simulink model "IPMSMAxleDriveEV_fihPedals"  (R2024a)
settings: Solver=FixedStepDiscrete  StartTime=0.0  StopTime=5  FixedStep=Ts  RelTol=1e-3  EnableMultiTasking=on
PreLoadFcn:
  | IPMSMAxleDriveEVData;
undefined symbols (not defined in the file): AL, Cd, cr1, cr2, g, i_t, Ld, Lq, Mv, p, psim, rho_a, Rw, Tmax, Ts, VDC_VECT
libraries: fl_lib x40, nesl_utility x16, ee_lib x4, eeTransforms x2, simulink x2, batteryecm_lib x1, eePmsmCurrentController x1, eePmsmCurrentReferenceGen x1, eePmsmTorqueEstimator x1, eePwmGeneratorTwoLevel x1, SignalEditorBlockLib x1
CloseFcn:
  | try,close(h1_IPMSMAxleDriveEV),end
  | clear h1_IPMSMAxleDriveEV
  | 
  | clear simlog_IPMSMAxleDriveEV
  | clear logsout_IPMSMAxleDriveEV
  | 
  | 
  | clear Pmax Tmax p psim Ld Lq L0 Rs Jm
  | clear Cdc Vnom V1 AH0
  | clear Ts fsw Tsi Kp_id Ki_id Kp_iq Ki_iq
  | clear numd_id dend_id numd_iq dend_iq
  | clear ID_MAP IQ_MAP RPM_VECT TQ_VECT VDC_VECT
  | clear Mv g rho_a AL Cd cr1 cr2 i_t Rw
Description:
  | IPMSM Torque Control in an Axle-Drive EV
settings Model: Creator=The MathWorks, Inc.  LastModifiedBy=hirah
settings SolverCC: AlgebraicLoopSolver=TrustRegion  MaxZcPerStep=1
settings DataIOCC: MaxDataPoints=510000  ReturnWorkspaceOutputs=off  SignalLoggingName=logsout_IPMSMAxleDriveEV
settings OptimizationCC: ReuseModelBlockBuffer=off  LifeSpan=inf
settings DebuggingCC: UnderspecifiedInitializationDetection=Classic  MergeDetectMultiDrivingBlocksExec=none  UnconnectedInputMsg=warning  UnconnectedOutputMsg=warning  UnconnectedLineMsg=warning  SFUnexpectedBacktrackingDiag=warning  SFNoUnconditionalDefaultTransitionDiag=warning  SFExecutionAtInitializationDiag=none  ArithmeticOperatorsInVariantConditions=warning
settings ModelReferenceCC: EnableRefExpFcnMdlSchedulingChecks=on
settings SFSimCC: SimUseLocalCustomCode=off  CustomCodeUndefinedFunction=UseInterfaceOnly
settings RTWCC: RTWUseLocalCustomCode=off  GPUComputeCapability=3.5  DLArmComputeVersion=19.05
settings CodeAppCC: StateflowObjectComments=on
settings GRTTargetCC: TargetLangStandard=C89/C90 (ANSI)
settings ConfigComp: CovMetricSettings=dw  CovSaveCumulativeToWorkspaceVar=on  CovSaveSingleToWorkspaceVar=on  CovExternalEMLEnable=off
settings SimscapeCC: SimscapeNormalizeSystem=off  SimscapeLogType=all  SimscapeLogSimulationStatistics=on  SimscapeLogName=simlog_IPMSMAxleDriveEV  SimscapeLogDataHistory=510000

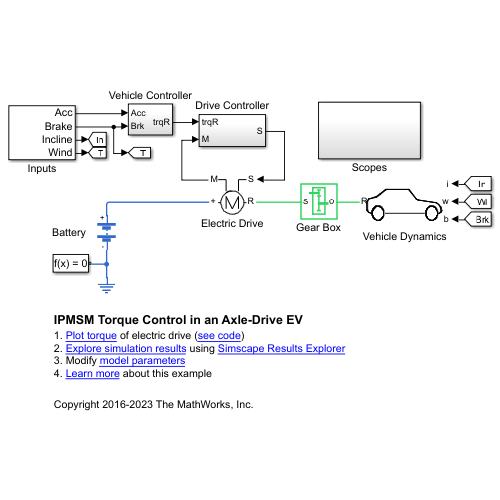
[thumbnail: Simulink's stored preview of the top-level diagram]
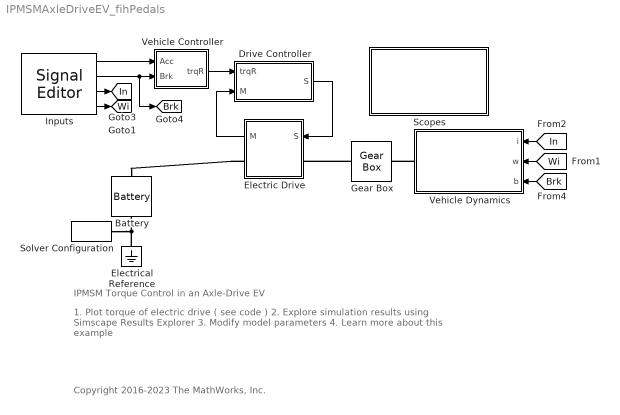
== system IPMSMAxleDriveEV_fihPedals ==
  note: IPMSM Torque Control in an Axle-Drive EV
  note: 1. Plot torque of electric drive ( see code )
      | 2. Explore simulation results using Simscape Results Explorer
      | 3. Modify model parameters
      | 4. Learn more about this example
  note: Copyright 2016-2023 The MathWorks, Inc.
  Battery : batteryecm_lib/Battery  Vnom=Vnom V  prm_dir=1  R1_dis=2 Ohm  R1_ch=2 Ohm  R1=0.001 Ohm  prm_AH=1  AH=300 hr*A  V1=V1 V  AH1=100 hr*A  prm_R2=1  R2=2000 Ohm  Tmeas=298.15 K  charge_measurement_port=simscape.enum.battery.enable.no  prm_dyn=1  Rp1=0.005 Ohm  tau1=30 s  Rp2=0.005 Ohm  tau2=30 s  Rp3=0.005 Ohm  tau3=30 s  Rp4=0.005 Ohm  tau4=30 s  Rp5=0.005 Ohm  tau5=30 s  prm_fade=1  N_fade=100  AH_fade=45 hr*A  R1_fade=2.02 Ohm  R1_ch_fade=2.02 Ohm  V1_fade=10.35 V  prm_age=1  prm_age_OCV=1  OCV_age=0.9  SOC_age=60  Tmeas_age=298.15 K  delta_time_age_vec=[0] d  temperature_age_vec=[273] K  OCV_scaling_age=2.2134e6  OCV_offset_age=1.632e6  temp_exp_age=0.515833569 V  t_exp_age=0.75  Vnom_T2=12 V  R1_T2=2.2 Ohm  R1_T2_dis=2.2 Ohm  R1_T2_ch=2.2 Ohm  V1_T2=11.4 V  R2_T2=2200 Ohm  Rp1_T2=0.005 Ohm  tau1_T2=30 s  Rp2_T2=0.005 Ohm  tau2_T2=30 s  Rp3_T2=0.005 Ohm  tau3_T2=30 s  Rp4_T2=0.005 Ohm  tau4_T2=30 s  Rp5_T2=0.005 Ohm  tau5_T2=30 s  Tmeas2=273.15 K  thermal_port=simscape.enum.thermaleffects.omit  thermal_mass=30000 J/K  i_specify=off  i_priority=None  i=0 A  i_nominal_specify=off  i_nominal_value=1  i_nominal_unit=A  v_specify=off  v_priority=None  v=0 V  v_nominal_specify=off  v_nominal_value=1  v_nominal_unit=V  charge_specify=on  charge_priority=High  charge=AH0 hr*A  charge_nominal_specify=off  charge_nominal_value=1  charge_nominal_unit=A*hr  num_cycles_specify=off  num_cycles_priority=High  num_cycles=0  num_cycles_nominal_specify=off  num_cycles_nominal_value=1  num_cycles_nominal_unit=1  temperature_specify=off  temperature_priority=High  temperature=298.15 K  temperature_nominal_specify=off  temperature_nominal_value=1  temperature_nominal_unit=K
  Drive Controller : Subsystem
  Electric Drive : Subsystem  Tag=PublishSubsystem
      mask Display:
      | % Circle
      | plot(sin(0:0.1:2.2*pi)*0.9,cos(0:0.1:2.2*pi)*0.9);
      | 
      | % In/out
      | plot([-1.1 -0.9],[0 0]);
      | plot([1.1 0.9],[0 0]);
      | 
      | % 'M'
      | plot([0.5 0.5],[-0.5 0.5]);
      | plot([-0.5 -0.5],[-0.5 0.5]);
      | plot([0.5 0],[0.5 -0.5]);
      | plot([-0.5 0],[0.5 -0.5]);
      | 
      | % Inputs and Outputs
      | plot([0.5 0.5],[0.9 1.8]);
      | plot([0.5 1.1],[1.8 1.8]);
      | 
      | plot([-0.5 -0.5],[0.9 1.8]);
      | plot([-0.5 -1.1],[1.8 1.8]);
      | 
      | 
      | % Plot points to set plot range
      | color('white');plot(1.9,2.8);plot(-1.9,0)
      | color('black');
  Electrical Reference : fl_lib/Electrical/Electrical Elements/Electrical Reference
  Gear Box : fl_lib/Mechanical/Mechanisms/Gear Box  ratio=i_t  t_in_specify=off  t_in_priority=None  t_in=0 N*m  t_in_nominal_specify=off  t_in_nominal_value=1  t_in_nominal_unit=N*m  t_out_specify=off  t_out_priority=None  t_out=0 N*m  t_out_nominal_specify=off  t_out_nominal_value=1  t_out_nominal_unit=N*m
  Inputs : SignalEditorBlockLib/Signal Editor  FileName=IPMSMAxleDriveEVInputs.mat  ActiveScenario=StartStop  ActiveSignal=Wind  IsBus=off  OutputBusObjectStr=Bus: BusObject  SampleTime=0  OutputAfterFinalValue=Extrapolation  Unit=inherit  PreserveSignalName=on  ApplySigPropsToAllScenarios=on  ApplySigPropsToAllSignals=off
  Scopes : Subsystem
  Solver Configuration : nesl_utility/Solver Configuration  PhysicalDomain=network_engine_domain  SubClassName=solver  LeftPortType=input  RightPortType=generic  Tones=[]  Harmonics=[]  SimulateNoise=off  Profile=off  UseLocalSampling=off  EnableSwitchedLinearOptims=on  FrequencyDomain=off  UseCCode=off  RelTol=0.001  AbsTol=1e-06  MinStep=1e-09  ToWorkspace=off  RevertToSquareIcSolve=off  NumHomotopyIterations=100  PhasorMode=off  PhasorModeNumHarmonics=1  ConsistencySolver=NEWTON_FTOL  IndexReductionMethod=DerivativeReplacement  DoDC=off  ResidualTolerance=1e-9  ConsistencyTolSource=GLOBAL  ConsistencyAbsTol=0.001  ConsistencyRelTol=0.001  ConsistencyTolFactor=0.001  UseLocalSolver=on  LocalSolverChoice=NE_BACKWARD_EULER_ADVANCER  ResolveIndetEquations=on  FunctionEvalNumThread=1  LocalSolverSampleTime=Ts  DoFixedCost=on  MaxNonlinIter=5  MaxModeIter=2  ComputeImpulses=off  ImpulseIterations=1  LinearAlgebra=auto  LinearAlgebraNumThread=0  EquationFormulation=NE_TIME_EF  DelaysMemoryBudget=1024  AutomaticFiltering=on  FilteringTimeConstant=0.001  PartitionStorageMethod=AS_NEEDED  PartitionMemoryBudget=1024  PartitionMethod=FAST  MultibodyUseLocalSolver=off  MultibodyLocalSolverChoice=ODE1  MultibodyLocalSolverSampleTime=0.001
  Vehicle Controller : Subsystem
  Vehicle Dynamics : Subsystem
      mask Display:
      | color('white')
      | plot(-120,-60); plot(120,50);
      | color('black')
      | plot(sin(0:0.1:6*pi)*15-70,cos(0:0.1:6*pi)*15-30);
      | plot(sin(0:0.1:6*pi)*15+70,cos(0:0.1:6*pi)*15-30);
      | plot([-88 -95 -99 -99 -95 -75 -65 -50 -46 10 30 34 80 85 90 93 95 93 90 88],[-30 -28 -23 -5 0 5 10 20 21 21 0 -2 -7 -9 -13 -17 -25 -28 -30 -30])
      | plot([-88 -95 -99 -99 -95 -75 -65 -50 -46 10 30 34 80 85 90 93 95 93 90 88],[-30 -28 -23 -5 0 5 10 20 21 21 0 -2 -7 -9 -13 -17 -25 -28 -30 -30]-1)
      | plot([-88 -95 -99 -99 -95 -75 -65 -50 -46 10 30 34 80 85 90 93 95 93 90 88]+1,[-30 -28 -23 -5 0 5 10 20 21 21 0 -2 -7 -9 -13 -17 -25 -28 -30 -30])
      | plot([-50 50],[-30 -30])
  tag scope: Brk=global, In=global, Wi=global
  wires:
  Vehicle Controller/1(trqR) -> Drive Controller/1(trqR)
  Electric Drive/1(M) -> Drive Controller/2(M)
  [Wi] -> Vehicle Dynamics/2(w)
  Drive Controller/1(S) -> Electric Drive/1(S)
  Inputs/3 -> [In]
  [Brk] -> Vehicle Dynamics/3(b)
  [In] -> Vehicle Dynamics/1(i)
  Inputs/1 -> Vehicle Controller/1(Acc)
  Inputs/2 -> [Brk], Vehicle Controller/2(Brk)
  Inputs/4 -> [Wi]
  connections:
  Battery/RConn1 -- Electrical Reference/LConn1 -- Solver Configuration/RConn1
  Electric Drive/RConn1 -- Battery/LConn1
  Gear Box/LConn1 -- Electric Drive/LConn1
  Vehicle Dynamics/RConn1 -- Gear Box/RConn1

== system IPMSMAxleDriveEV_fihPedals/Drive Controller ==
  trqR : Inport
  M : Inport  Port=2
  Bus Selector : BusSelector  OutputSignals=iabc,w,A,vdc
  EM Controller : Subsystem
  S : Outport  VectorParamsAs1DForOutWhenUnconnected=off
  wires:
  M/1 -> Bus Selector/1
  trqR/1 -> EM Controller/1(trqR)
  Bus Selector/1 -> EM Controller/2(iabc_sens)  "<iabc>"
  Bus Selector/2 -> EM Controller/3(w_sens)  "<w>"
  Bus Selector/3 -> EM Controller/4(th_sens)  "<A>"
  Bus Selector/4 -> EM Controller/5(Vdc_sens)  "<vdc>"
  EM Controller/1(S) -> S/1

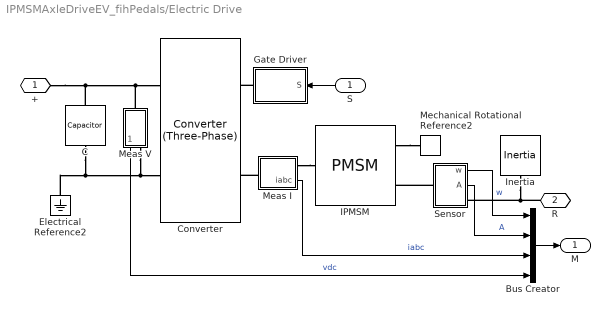
== system IPMSMAxleDriveEV_fihPedals/Electric Drive ==
  S : Inport
  Bus Creator : BusCreator  Inputs=4
  C : fl_lib/Electrical/Electrical Elements/Capacitor  c=Cdc F  r=1e-6 Ohm  g=0 1/Ohm  i_specify=off  i_priority=None  i=0 A  i_nominal_specify=off  i_nominal_value=1  i_nominal_unit=A  v_specify=off  v_priority=None  v=0 V  v_nominal_specify=off  v_nominal_value=1  v_nominal_unit=V  vc_specify=on  vc_priority=None  vc=Vnom V  vc_nominal_specify=off  vc_nominal_value=1  vc_nominal_unit=V
  Converter : ee_lib/Semiconductors & Converters/Converters/Converter (Three-Phase)  port_option=ee.enum.threePhasePort.composite  fidelity_option=ee.enum.converters.fidelity.detailed  device_type=3  K=0  Vf=0.8 V  Ron=0.001 Ohm  Rds=0.001 Ohm  Goff=1e-5 1/Ohm  Vgt=1 V  Vgt_off=-1 V  Ih=1 A  Vth=0.5 V  diode_param=2  diode_Vf=0.8 V  diode_Ron=0.001 Ohm  diode_Goff=1e-5 1/Ohm  diode_C=50 nF  diode_iRM=-235 A  diode_iF=300 A  diode_idot=-50 A/us  diode_trr_param=1  diode_trr_factor=3  diode_trr=15 us  diode_Qrr=1.5e+3 s*uA  snubber_type=0  Cs=1e-7 F  Rs=0.1 Ohm
  Electrical Reference2 : fl_lib/Electrical/Electrical Elements/Electrical Reference
  Gate Driver : Subsystem
  IPMSM : ee_lib/Electromechanical/Permanent Magnet/PMSM  port_option=ee.enum.threePhasePort.composite  winding_type=ee.enum.statorconnection.wye  machine_param=ee.enum.pmsm.parameterization.constant  nPolePairs=p  pmflux_param=1  pm_flux_linkage=psim Wb  torque_constant=0.18 N*m/A  back_emf_constant=0.18 V/(rad/s)  stator_param=1  Ld=Ld H  Lq=Lq H  idVec=[-200, 0, 200] A  iqVec=[-200, 0, 200] A  LdMatrix=0.0002 * ones(3, 3) H  LqMatrix=0.0002 * ones(3, 3) H  PmMatrix=0.1 * ones(3, 3) Wb  ktMatrix=0.18 * ones(3, 3) N*m/A  keMatrix=0.18 * ones(3, 3) V/(rad/s)  L0=L0 H  Ls=0.0002 H  Lm=0.00002 H  Ms=0.00002 H  Rs=Rs Ohm  zero_sequence=ee.enum.park.zerosequence.exclude  axes_param=1  loss_param=ee.enum.ironloss.none  losses_oc=[0, 0, 0] W  losses_sc=[0, 0, 0] W  f_losses=60 Hz  Isc_losses=95 A  J=0 kg*m^2  lam=0 N*m/(rad/s)  i_d_specify=off  i_d_priority=None  i_d=0 A  i_d_nominal_specify=off  i_d_nominal_value=1  i_d_nominal_unit=A  i_q_specify=off  i_q_priority=None  i_q=0 A  i_q_nominal_specify=off  i_q_nominal_value=1  i_q_nominal_unit=A  torque_specify=off  torque_priority=None  torque=0 N*m  torque_nominal_specify=off  torque_nominal_value=1  torque_nominal_unit=N*m  angular_velocity_specify=on  angular_velocity_priority=None  angular_velocity=0 rpm  angular_velocity_nominal_specify=off  angular_velocity_nominal_value=1  angular_velocity_nominal_unit=rpm  angular_position_specify=off  angular_position_priority=None  angular_position=0 deg  angular_position_nominal_specify=off  angular_position_nominal_value=1  angular_position_nominal_unit=deg  alpha=3.93e-3 1/K  alpha_flux=-0.001 1/K  Tmeas=298.15 K  stator_thermal_mass=100 J/K  rotor_thermal_mass=200 J/K  Rm_percent_rotor=90  Rd_percent_rotor=30  temperatureA_specify=off  temperatureA_priority=High  temperatureA=25 degC  temperatureA_nominal_specify=off  temperatureA_nominal_value=1  temperatureA_nominal_unit=degC  temperatureB_specify=off  temperatureB_priority=High  temperatureB=25 degC  temperatureB_nominal_specify=off  temperatureB_nominal_value=1  temperatureB_nominal_unit=degC  temperatureC_specify=off  temperatureC_priority=High  temperatureC=25 degC  temperatureC_nominal_specify=off  temperatureC_nominal_value=1  temperatureC_nominal_unit=degC  temperatureR_specify=off  temperatureR_priority=High  temperatureR=25 degC  temperatureR_nominal_specify=off  temperatureR_nominal_value=1  temperatureR_nominal_unit=degC
      settings: AttributesFormatString=35 kW  InternalSimscapePortConfiguration="{\"Bottom\":[],\"Left\":[{\"id\":\"N\",\"label\":\"~\",\"type\":\"foundation.electrical.three_phase\"}],\"Right\":[{\"id\":\"R\",\"label\":\"R\",\"type\":\"foundation.mechanical.rotational.rotational\"},{\"id\":\"C\",\"label\":\"C\",\"type\":\"foundation.mechanical.rotational.rotational\"}],\"Top\":[]}"
  Inertia : fl_lib/Mechanical/Rotational Elements/Inertia  inertia=Jm kg*m^2  num_ports=foundation.enum.numPorts2.one  w_specify=off  w_priority=High  w=0 rad/s  w_nominal_specify=off  w_nominal_value=1  w_nominal_unit=rad/s  t_specify=off  t_priority=None  t=0 N*m  t_nominal_specify=off  t_nominal_value=1  t_nominal_unit=N*m
  Meas I : Subsystem
      settings: PortSchema="{\"entries\":[{\"content\":{\"sides\":[{\"content\":{\"connectorIds\":[\"LConn1\"]},\"type\":\"ConnectorPlacement.EquallySpacedRectSide\",\"uuid\":\"3a4028b2-8937-42a6-80f4-68b1695ce77d\"},{\"content\":{\"connectorIds\":[\"RConn1\",\"Out1\"],\"side\":\"RIGHT\"},\"type\":\"ConnectorPlacement.EquallySpacedRectSide\",\"uuid\":\"b0265b90-0b10-444b-91c2-8367167e2f75\"},{\"content\":{\"connectorIds\":[],\"side\":\"TOP\"},\"type\":\"ConnectorPlacement.EquallySpacedRectSide\",\"uuid\":\"a56d3a18-e083-4f19-8a6c-1d5eb0dcfc62\"}]},\"type\":\"ConnectorPlacement.EquallySpacedConnector\",\"uuid\":\"f333dc84-7c1b-47f0-a9ed-bc0e1c61b934\"}],\"packageUris\":[\"http://schema.mathworks.com/mf0/Connector/R2020b\"],\"version\":\"1.0\"}"
      mask Display: %disp('iABC');
  Meas V : Subsystem
  Mechanical Rotational Reference2 : fl_lib/Mechanical/Rotational Elements/Mechanical Rotational Reference
  Sensor : Subsystem
  + : PMIOPort  Side=Right
  R : PMIOPort  Port=2  Side=Left
  M : Outport  VectorParamsAs1DForOutWhenUnconnected=off
  wires:
  S/1 -> Gate Driver/1(S)
  Bus Creator/1 -> M/1
  Meas I/1(iabc) -> Bus Creator/3  "iabc"
  Sensor/1(w) -> Bus Creator/1  "w"
  Sensor/2(A) -> Bus Creator/2  "A"
  Meas V/1(Vdc) -> Bus Creator/4  "vdc"
  connections:
  Gate Driver/RConn1 -- Converter/LConn1
  IPMSM/RConn2 -- Mechanical Rotational Reference2/LConn1
  Meas I/LConn1 -- Converter/LConn2
  Sensor/LConn1 -- IPMSM/RConn1
  Meas I/RConn1 -- IPMSM/LConn1
  R/RConn1 -- Sensor/RConn1 -- Inertia/LConn1
  +/RConn1 -- C/LConn1 -- Meas V/LConn1 -- Converter/RConn1
  Electrical Reference2/LConn1 -- C/RConn1 -- Meas V/RConn1 -- Converter/RConn2

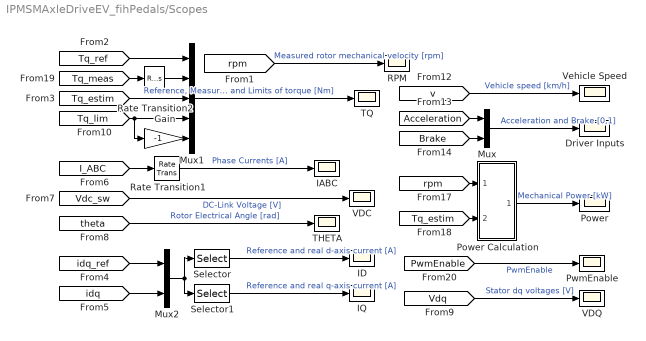
== system IPMSMAxleDriveEV_fihPedals/Scopes ==
  Driver Inputs : Scope
  Gain : Gain  Gain=-1
  IABC : Scope
  ID : Scope
  IQ : Scope
  Mux : Mux  Inputs=2
  Mux1 : Mux  Inputs=5
  Mux2 : Mux  Inputs=2
  Power : Scope
  Power Calculation : Subsystem
  PwmEnable : Scope
  RPM : Scope
  Rate Transition1 : RateTransition  OutPortSampleTime=1e-4
  Rate Transition2 : RateTransition
  Selector : Selector  InputPortWidth=4  IndexOptions=Index vector (dialog)  Indices=[1 3]  OutputSizes=1
  Selector1 : Selector  InputPortWidth=4  IndexOptions=Index vector (dialog)  Indices=[2 4]  OutputSizes=1
  THETA : Scope
  TQ : Scope
  VDC : Scope
  VDQ : Scope
  Vehicle Speed : Scope
  wires:
  Power Calculation/1(Power) -> Power/1  "Mechanical Power [kW]"
  Gain/1 -> Mux1/5
  [idq] -> Mux2/2
  [Tq_meas] -> Rate Transition2/1
  [Tq_estim] -> Mux1/3
  [rpm] -> Power Calculation/1(rpm)
  [Tq_estim] -> Power Calculation/2(Tq)
  [idq_ref] -> Mux2/1
  [v] -> Vehicle Speed/1  "Vehicle speed [km/h]"
  Mux1/1 -> TQ/1  "Reference, Measured, Estim and Limits of torque [Nm]"
  [Vdq] -> VDQ/1  "Stator dq voltages [V]"
  [I_ABC] -> Rate Transition1/1
  [Tq_ref] -> Mux1/1
  [Tq_lim] -> Gain/1, Mux1/4
  [PwmEnable] -> PwmEnable/1  "PwmEnable"
  Rate Transition2/1 -> Mux1/2
  [theta] -> THETA/1  "Rotor Electrical Angle [rad]"
  Selector/1 -> ID/1  "Reference and real d-axis current [A]"
  Mux2/1 -> Selector1/1, Selector/1
  Mux/1 -> Driver Inputs/1  "Acceleration and Brake [0,1]"
  Selector1/1 -> IQ/1  "Reference and real q-axis current [A]"
  [Brake] -> Mux/2
  [Acceleration] -> Mux/1
  Rate Transition1/1 -> IABC/1  "Phase Currents [A]"
  [rpm] -> RPM/1  "Measured rotor mechanical velocity [rpm]"
  [Vdc_sw] -> VDC/1  "DC-Link Voltage [V]"

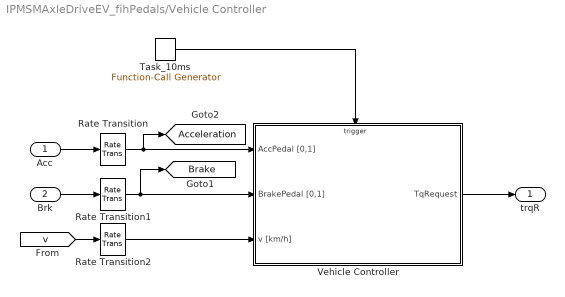
== system IPMSMAxleDriveEV_fihPedals/Vehicle Controller ==
  Acc : Inport
  Brk : Inport  Port=2
  Rate Transition : RateTransition
  Rate Transition1 : RateTransition
  Rate Transition2 : RateTransition
  Task_10ms : simulink/Ports & Subsystems/Function-Call Generator  sample_time=0.01  numberOfIterations=1  DisallowWideOutput=off
  Vehicle Controller : Subsystem
  trqR : Outport  VectorParamsAs1DForOutWhenUnconnected=off
  tag scope: Acceleration=global, Brake=global
  wires:
  Acc/1 -> Rate Transition/1
  Task_10ms/1 -> Vehicle Controller/Trigger
  Vehicle Controller/1(TqRequest) -> trqR/1
  Brk/1 -> Rate Transition1/1
  Rate Transition/1 -> Vehicle Controller/1(AccPedal [0,1]), [Acceleration]
  Rate Transition1/1 -> [Brake], Vehicle Controller/2(BrakePedal [0,1])
  [v] -> Rate Transition2/1
  Rate Transition2/1 -> Vehicle Controller/3(v [km/h])

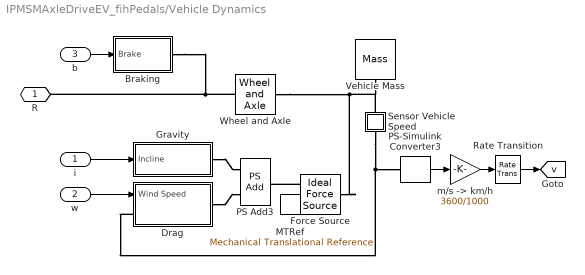
== system IPMSMAxleDriveEV_fihPedals/Vehicle Dynamics ==
  i : Inport
  w : Inport  Port=2
  b : Inport  Port=3
  Braking : Subsystem
  Drag : Subsystem
  Force Source : fl_lib/Mechanical/Mechanical Sources/Ideal Force Source
  Gravity : Subsystem
  MTRef : fl_lib/Mechanical/Translational Elements/Mechanical Translational Reference
  PS Add3 : fl_lib/Physical Signals/Functions/PS Add
  PS-Simulink Converter3 : nesl_utility/PS-Simulink Converter  PhysicalDomain=network_engine_domain  SubClassName=ps_output  LeftPortType=input  RightPortType=output  PseudoPeriodic=off  Frequencies=[]  VectorFormat=1-D array  Unit=m/s  AffineConversion=off
  Rate Transition : RateTransition  OutPortSampleTime=1e-4
  Sensor Vehicle Speed : Subsystem
      mask Display: disp('v')
  Vehicle Mass : fl_lib/Mechanical/Translational Elements/Mass  mass=Mv kg  num_ports=foundation.enum.numPorts2.one  v_specify=off  v_priority=High  v=0 m/s  v_nominal_specify=off  v_nominal_value=1  v_nominal_unit=m/s  f_specify=off  f_priority=None  f=0 N  f_nominal_specify=off  f_nominal_value=1  f_nominal_unit=N
  Wheel and Axle : fl_lib/Mechanical/Mechanisms/Wheel and Axle  R=Rw m  or=1  t_specify=off  t_priority=None  t=0 N*m  t_nominal_specify=off  t_nominal_value=1  t_nominal_unit=N*m  f_specify=off  f_priority=None  f=0 N  f_nominal_specify=off  f_nominal_value=1  f_nominal_unit=N
  "m/s -> km/h" : Gain  Gain=3600/1000
  R : PMIOPort  Side=Right
  tag scope: v=global
  wires:
  PS-Simulink Converter3/1 -> "m/s -> km/h"/1
  "m/s -> km/h"/1 -> Rate Transition/1
  Rate Transition/1 -> [v]
  b/1 -> Braking/1(Brake)
  w/1 -> Drag/1(Wind Speed)
  i/1 -> Gravity/1(Incline)
  connections:
  Wheel and Axle/LConn1 -- Braking/RConn1 -- R/RConn1
  MTRef/LConn1 -- Force Source/RConn2
  Drag/RConn1 -- PS Add3/LConn2
  Gravity/RConn1 -- PS Add3/LConn1
  Force Source/RConn1 -- PS Add3/RConn1
  Drag/LConn1 -- Sensor Vehicle Speed/RConn1 -- PS-Simulink Converter3/LConn1
  Wheel and Axle/RConn1 -- Vehicle Mass/LConn1 -- Sensor Vehicle Speed/LConn1 -- Force Source/LConn1

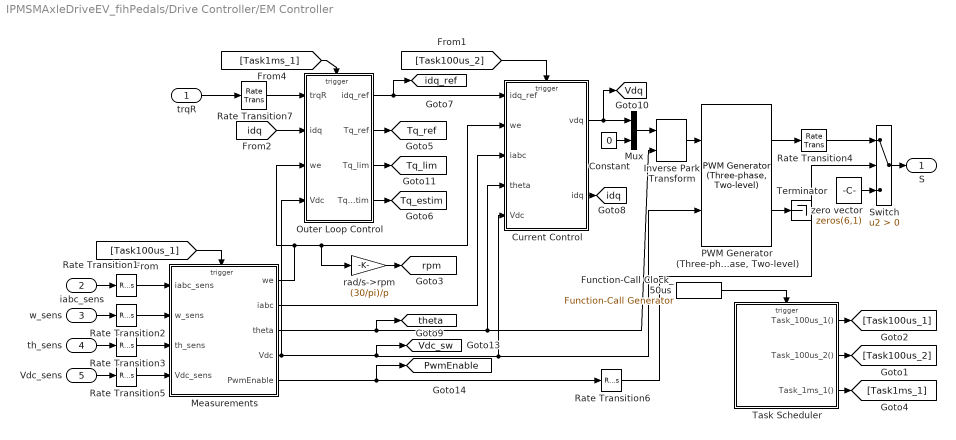
== system IPMSMAxleDriveEV_fihPedals/Drive Controller/EM Controller ==
  trqR : Inport
  iabc_sens : Inport  Port=2
  w_sens : Inport  Port=3
  th_sens : Inport  Port=4
  Vdc_sens : Inport  Port=5
  Constant : Constant  Value=0  SampleTime=-1
  Current Control : Subsystem
  Function-Call Clock_50us : simulink/Ports & Subsystems/Function-Call Generator  sample_time=5e-5  numberOfIterations=1  DisallowWideOutput=off
  Inverse Park Transform : eeTransforms/Inverse Park Transform  AxisAlignment=Q-axis  PowerInvariant=off
  Measurements : Subsystem
  Mux : Mux  Inputs=2
  Outer Loop Control : Subsystem
  "PWM Generator (Three-phase, Two-level)" : eePwmGeneratorTwoLevel/PWM Generator (Three-phase, Two-level)  PWMMode=Continuous PWM (CPWM)  CPWMMode=SVM: space vector modulation  DPWMMode=60 DPWM: 60 degree discontinuous PWM  fsw=fsw  Ts=Ts
  Rate Transition{1..7} (7 alike) : RateTransition
  Switch : Switch  Criteria=u2 > Threshold  SaturateOnIntegerOverflow=off  InputSameDT=off
  Task Scheduler : Stateflow chart  TreatAsAtomicUnit=on
  Terminator : Terminator
  rad/s->rpm : Gain  Gain=(30/pi)/p
  zero vector : Constant  Value=zeros(6,1)
  S : Outport  VectorParamsAs1DForOutWhenUnconnected=off
  tag scope: PwmEnable=global, Tq_estim=global, Tq_lim=global, Tq_ref=global, Vdc_sw=global, Vdq=global, idq=global, idq_ref=global, rpm=global, theta=global
  wires:
  Measurements/5(PwmEnable) -> [PwmEnable], Rate Transition6/1
  Current Control/1(vdq) -> [Vdq], Mux/1
  [Task100us_2] -> Current Control/Trigger
  Rate Transition7/1 -> Outer Loop Control/1(trqR)
  Function-Call Clock_50us/1 -> Task Scheduler/Trigger
  Task Scheduler/2(Task_100us_2()) -> [Task100us_2]
  [idq] -> Outer Loop Control/2(idq)
  "PWM Generator (Three-phase, Two-level)"/2 -> Terminator/1
  Rate Transition3/1 -> Measurements/3(th_sens)
  Rate Transition6/1 -> Switch/2
  Task Scheduler/3(Task_1ms_1()) -> [Task1ms_1]
  Inverse Park Transform/1 -> "PWM Generator (Three-phase, Two-level)"/1
  "PWM Generator (Three-phase, Two-level)"/1 -> Rate Transition4/1
  Outer Loop Control/3(Tq_lim) -> [Tq_lim]
  trqR/1 -> Rate Transition7/1
  Vdc_sens/1 -> Rate Transition5/1
  Measurements/4(Vdc) -> Outer Loop Control/4(Vdc), Current Control/5(Vdc), "PWM Generator (Three-phase, Two-level)"/2, [Vdc_sw]
  Measurements/1(we) -> Outer Loop Control/3(we), rad/s->rpm/1, Current Control/2(we)
  Rate Transition5/1 -> Measurements/4(Vdc_sens)
  rad/s->rpm/1 -> [rpm]
  Measurements/3(theta) -> [theta], Inverse Park Transform/2, Current Control/4(theta)
  Outer Loop Control/2(Tq_ref) -> [Tq_ref]
  iabc_sens/1 -> Rate Transition1/1
  Current Control/2(idq) -> [idq]
  th_sens/1 -> Rate Transition3/1
  Rate Transition2/1 -> Measurements/2(w_sens)
  Outer Loop Control/4(Tq_estim) -> [Tq_estim]
  Rate Transition4/1 -> Switch/1
  Outer Loop Control/1(idq_ref) -> Current Control/1(idq_ref), [idq_ref]
  Switch/1 -> S/1
  w_sens/1 -> Rate Transition2/1
  Task Scheduler/1(Task_100us_1()) -> [Task100us_1]
  Rate Transition1/1 -> Measurements/1(iabc_sens)
  [Task1ms_1] -> Outer Loop Control/Trigger
  [Task100us_1] -> Measurements/Trigger
  zero vector/1 -> Switch/3
  Measurements/2(iabc) -> Current Control/3(iabc)
  Mux/1 -> Inverse Park Transform/1
  Constant/1 -> Mux/2

== system IPMSMAxleDriveEV_fihPedals/Electric Drive/Gate Driver ==
  S : Inport
  Demux : Demux  Outputs=6
  Simulink-PS Converter{1..6} (6 alike) : nesl_utility/Simulink-PS Converter  PhysicalDomain=network_engine_domain  SubClassName=ps_input  LeftPortType=input  RightPortType=output  PseudoPeriodic=off  Frequencies=[]  NoiseDistribution=none  NoiseParameters=[]  Unit=1  AffineConversion=off  FilteringAndDerivatives=zero  SimscapeFilterOrder=1  InputFilterTimeConstant=0.001  UdotUserProvided=1
  Six-Pulse Gate Multiplexer : ee_lib/Semiconductors & Converters/Converters/Six-Pulse Gate Multiplexer  port_option=ee.enum.controlport.ps
  G : PMIOPort  Side=Right
  wires:
  Demux/1 -> Simulink-PS Converter1/1
  S/1 -> Demux/1
  Demux/4 -> Simulink-PS Converter4/1
  Demux/2 -> Simulink-PS Converter2/1
  Demux/3 -> Simulink-PS Converter3/1
  Demux/5 -> Simulink-PS Converter5/1
  Demux/6 -> Simulink-PS Converter6/1
  connections:
  Six-Pulse Gate Multiplexer/RConn1 -- G/RConn1
  Simulink-PS Converter1/RConn1 -- Six-Pulse Gate Multiplexer/LConn1
  Simulink-PS Converter3/RConn1 -- Six-Pulse Gate Multiplexer/LConn3
  Simulink-PS Converter5/RConn1 -- Six-Pulse Gate Multiplexer/LConn5
  Simulink-PS Converter6/RConn1 -- Six-Pulse Gate Multiplexer/LConn6
  Simulink-PS Converter4/RConn1 -- Six-Pulse Gate Multiplexer/LConn4
  Simulink-PS Converter2/RConn1 -- Six-Pulse Gate Multiplexer/LConn2

== system IPMSMAxleDriveEV_fihPedals/Electric Drive/Meas I ==
  Current Sensor : ee_lib/Sensors & Transducers/Current Sensor (Three-Phase)
  PS-Simulink Converter : nesl_utility/PS-Simulink Converter  PhysicalDomain=network_engine_domain  SubClassName=ps_output  LeftPortType=input  RightPortType=output  PseudoPeriodic=off  Frequencies=[]  VectorFormat=1-D array  Unit=A  AffineConversion=off
  1 : PMIOPort  Side=Left
  2 : PMIOPort  Port=2  Side=Right
  iabc : Outport  VectorParamsAs1DForOutWhenUnconnected=off
  tag scope: I_ABC=global
  wires:
  PS-Simulink Converter/1 -> [I_ABC], iabc/1
  connections:
  1/RConn1 -- Current Sensor/LConn1
  2/RConn1 -- Current Sensor/RConn2
  Current Sensor/RConn1 -- PS-Simulink Converter/LConn1

== system IPMSMAxleDriveEV_fihPedals/Electric Drive/Meas V ==
  PS-Simulink Converter4 : nesl_utility/PS-Simulink Converter  PhysicalDomain=network_engine_domain  SubClassName=ps_output  LeftPortType=input  RightPortType=output  PseudoPeriodic=off  Frequencies=[]  VectorFormat=1-D array  Unit=V  AffineConversion=off
  Voltage Sensor : fl_lib/Electrical/Electrical Sensors/Voltage Sensor
  - : PMIOPort  Side=Right
  + : PMIOPort  Port=2  Side=Left
  Vdc : Outport  VectorParamsAs1DForOutWhenUnconnected=off
  wires:
  PS-Simulink Converter4/1 -> Vdc/1
  connections:
  PS-Simulink Converter4/LConn1 -- Voltage Sensor/RConn1
  Voltage Sensor/LConn1 -- +/RConn1
  Voltage Sensor/RConn2 -- -/RConn1

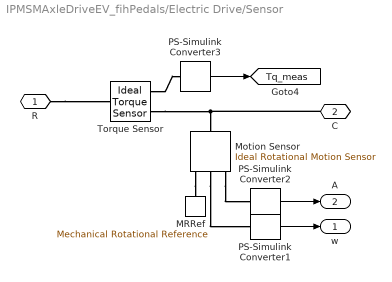
== system IPMSMAxleDriveEV_fihPedals/Electric Drive/Sensor ==
  MRRef : fl_lib/Mechanical/Rotational Elements/Mechanical Rotational Reference
  Motion Sensor : fl_lib/Mechanical/Mechanical Sensors/Ideal Rotational Motion Sensor  reference=foundation.enum.MeasurementReference.difference  acceleration_port=false  velocity_port=true  position_port=true  wrap_angle=simscape.enum.onoff.off  offset=0 deg
  PS-Simulink Converter1 : nesl_utility/PS-Simulink Converter  PhysicalDomain=network_engine_domain  SubClassName=ps_output  LeftPortType=input  RightPortType=output  PseudoPeriodic=off  Frequencies=[]  VectorFormat=1-D array  Unit=rad/s  AffineConversion=off
  PS-Simulink Converter2 : nesl_utility/PS-Simulink Converter  PhysicalDomain=network_engine_domain  SubClassName=ps_output  LeftPortType=input  RightPortType=output  PseudoPeriodic=off  Frequencies=[]  VectorFormat=1-D array  Unit=rad  AffineConversion=off
  PS-Simulink Converter3 : nesl_utility/PS-Simulink Converter  PhysicalDomain=network_engine_domain  SubClassName=ps_output  LeftPortType=input  RightPortType=output  PseudoPeriodic=off  Frequencies=[]  VectorFormat=1-D array  Unit=N*m  AffineConversion=off
  Torque Sensor : fl_lib/Mechanical/Mechanical Sensors/Ideal Torque Sensor
  R : PMIOPort  Side=Left
  C : PMIOPort  Port=2  Side=Right
  w : Outport  VectorParamsAs1DForOutWhenUnconnected=off
  A : Outport  Port=2  VectorParamsAs1DForOutWhenUnconnected=off
  tag scope: Tq_meas=global
  wires:
  PS-Simulink Converter3/1 -> [Tq_meas]
  PS-Simulink Converter1/1 -> w/1
  PS-Simulink Converter2/1 -> A/1
  connections:
  Motion Sensor/RConn2 -- PS-Simulink Converter1/LConn1
  Motion Sensor/RConn1 -- MRRef/LConn1
  R/RConn1 -- Torque Sensor/LConn1
  Torque Sensor/RConn1 -- C/RConn1 -- Motion Sensor/LConn1
  Torque Sensor/RConn2 -- PS-Simulink Converter3/LConn1
  Motion Sensor/RConn3 -- PS-Simulink Converter2/LConn1

== system IPMSMAxleDriveEV_fihPedals/Scopes/Power Calculation ==
  rpm : Inport
  Tq : Inport  Port=2
  Gain3 : Gain  Gain=pi/30
  Gain4 : Gain  Gain=1/1000
  Product2 : Product
  Power : Outport  VectorParamsAs1DForOutWhenUnconnected=off
  wires:
  rpm/1 -> Gain3/1
  Gain4/1 -> Power/1
  Product2/1 -> Gain4/1
  Tq/1 -> Product2/2
  Gain3/1 -> Product2/1

== system IPMSMAxleDriveEV_fihPedals/Vehicle Controller/Vehicle Controller ==
  AccPedal [0,1] : Inport
  BrakePedal [0,1] : Inport  Port=2
  v [km/h] : Inport  Port=3
  Task10ms : TriggerPort  TriggerType=function-call  VariantControl=Variant  PortDimensions=1
  Acceleration Pedal Characteristic : Lookup_n-D  NumberOfTableDimensions=1  BreakpointsForDimension1=0:0.1:1  Table=[0 0.04 0.07 0.1 0.16 0.2 0.3 0.4 0.6 0.8 1]*Tmax  InternalRulePriority=Speed  RndMeth=Simplest
  Brake Pedal Characteristic : Lookup_n-D  NumberOfTableDimensions=1  BreakpointsForDimension1=[0 0.03 0.04 0.3 0.4 0.5 0.6 0.7 0.8 0.9 1]  Table=[0 0 0.04 0.05 0.06 0.2 0.25 0.4 0.6 0.8 1]*(-Tmax)  InternalRulePriority=Speed  RndMeth=Simplest
  Constant : Constant  Value=0  SampleTime=-1
  Sum : Sum  Inputs=|++
  v>0 : Switch  Criteria=u2 > Threshold  Threshold=0.1  SaturateOnIntegerOverflow=off  InputSameDT=off
  TqRequest : Outport  VectorParamsAs1DForOutWhenUnconnected=off
  wires:
  AccPedal [0,1]/1 -> Acceleration Pedal Characteristic/1
  BrakePedal [0,1]/1 -> Brake Pedal Characteristic/1
  Acceleration Pedal Characteristic/1 -> Sum/1
  Sum/1 -> TqRequest/1
  Brake Pedal Characteristic/1 -> v>0/1
  Constant/1 -> v>0/3
  v>0/1 -> Sum/2
  v [km/h]/1 -> v>0/2

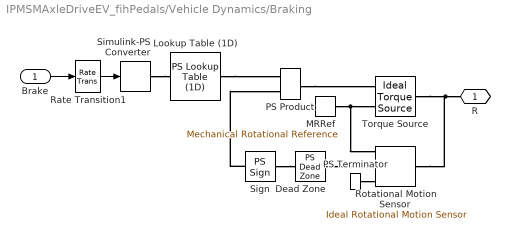
== system IPMSMAxleDriveEV_fihPedals/Vehicle Dynamics/Braking ==
  Brake : Inport
  Dead Zone : fl_lib/Physical Signals/Nonlinear Operators/PS Dead Zone  upper_limit=0.1 rad/s  lower_limit=-0.001 rad/s
      settings: InternalSimscapePortConfiguration="{\"Bottom\":[],\"Left\":[{\"id\":\"I\",\"label\":\"\",\"type\":\"input\"}],\"Right\":[{\"id\":\"O\",\"label\":\"\",\"type\":\"output\"}],\"Top\":[]}"
  Lookup Table (1D) : fl_lib/Physical Signals/Lookup Tables/PS Lookup Table (1D)  x=[0 0.03 0.04 0.3 0.4 0.5 0.6 0.7 0.8 0.9 1]  f=[0 0 0.04 0.05 0.06 0.2 0.25 0.4 0.6 0.8 1]*(-Tmax)*i_t N*m  interp_method=simscape.enum.interpolation.linear  extrap_method=simscape.enum.extrapolation.linear
  MRRef : fl_lib/Mechanical/Rotational Elements/Mechanical Rotational Reference
  PS Product : fl_lib/Physical Signals/Functions/PS Product
  PS Terminator : fl_lib/Physical Signals/Sinks/PS Terminator
  Rate Transition1 : RateTransition
  Rotational Motion Sensor : fl_lib/Mechanical/Mechanical Sensors/Ideal Rotational Motion Sensor  reference=foundation.enum.MeasurementReference.difference  acceleration_port=false  velocity_port=true  position_port=true  wrap_angle=simscape.enum.onoff.off  offset=0 rad
  Sign : fl_lib/Physical Signals/Nonlinear Operators/PS Sign
      settings: InternalSimscapePortConfiguration="{\"Bottom\":[],\"Left\":[{\"id\":\"I\",\"label\":\"\",\"type\":\"input\"}],\"Right\":[{\"id\":\"O\",\"label\":\"\",\"type\":\"output\"}],\"Top\":[]}"
  Simulink-PS Converter : nesl_utility/Simulink-PS Converter  PhysicalDomain=network_engine_domain  SubClassName=ps_input  LeftPortType=input  RightPortType=output  PseudoPeriodic=off  Frequencies=[]  NoiseDistribution=none  NoiseParameters=[]  Unit=1  AffineConversion=off  FilteringAndDerivatives=zero  SimscapeFilterOrder=1  InputFilterTimeConstant=0.001  UdotUserProvided=1
  Torque Source : fl_lib/Mechanical/Mechanical Sources/Ideal Torque Source
  R : PMIOPort  Side=Right
  wires:
  Brake/1 -> Rate Transition1/1
  Rate Transition1/1 -> Simulink-PS Converter/1
  connections:
  Torque Source/LConn1 -- Rotational Motion Sensor/LConn1 -- R/RConn1
  PS Product/RConn1 -- Torque Source/RConn1
  MRRef/LConn1 -- Rotational Motion Sensor/RConn1 -- Torque Source/RConn2
  PS Terminator/LConn1 -- Rotational Motion Sensor/RConn3
  Dead Zone/LConn1 -- Rotational Motion Sensor/RConn2
  Lookup Table (1D)/RConn1 -- PS Product/LConn1
  Sign/RConn1 -- PS Product/LConn2
  Simulink-PS Converter/RConn1 -- Lookup Table (1D)/LConn1
  Sign/LConn1 -- Dead Zone/RConn1

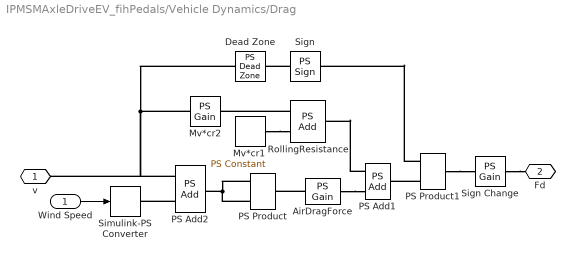
== system IPMSMAxleDriveEV_fihPedals/Vehicle Dynamics/Drag ==
  Wind Speed : Inport
  AirDragForce : fl_lib/Physical Signals/Functions/PS Gain  gain=0.5*rho_a*AL*Cd N/(m/s)^2
  Dead Zone : fl_lib/Physical Signals/Nonlinear Operators/PS Dead Zone  upper_limit=0.1 m/s  lower_limit=-0.001 m/s
      settings: InternalSimscapePortConfiguration="{\"Bottom\":[],\"Left\":[{\"id\":\"I\",\"label\":\"\",\"type\":\"input\"}],\"Right\":[{\"id\":\"O\",\"label\":\"\",\"type\":\"output\"}],\"Top\":[]}"
  Mv*cr1 : fl_lib/Physical Signals/Sources/PS Constant  constant=Mv*cr1 N
  Mv*cr2 : fl_lib/Physical Signals/Functions/PS Gain  gain=Mv*cr2 N/(m/s)
  PS Add1 : fl_lib/Physical Signals/Functions/PS Add
  PS Add2 : fl_lib/Physical Signals/Functions/PS Add
  PS Product : fl_lib/Physical Signals/Functions/PS Product
  PS Product1 : fl_lib/Physical Signals/Functions/PS Product
  RollingResistance : fl_lib/Physical Signals/Functions/PS Add
  Sign : fl_lib/Physical Signals/Nonlinear Operators/PS Sign
      settings: InternalSimscapePortConfiguration="{\"Bottom\":[],\"Left\":[{\"id\":\"I\",\"label\":\"\",\"type\":\"input\"}],\"Right\":[{\"id\":\"O\",\"label\":\"\",\"type\":\"output\"}],\"Top\":[]}"
  Sign Change : fl_lib/Physical Signals/Functions/PS Gain  gain=-1
  Simulink-PS Converter : nesl_utility/Simulink-PS Converter  PhysicalDomain=network_engine_domain  SubClassName=ps_input  LeftPortType=input  RightPortType=output  PseudoPeriodic=off  Frequencies=[]  NoiseDistribution=none  NoiseParameters=[]  Unit=m/s  AffineConversion=off  FilteringAndDerivatives=zero  SimscapeFilterOrder=1  InputFilterTimeConstant=0.001  UdotUserProvided=1
  v : PMIOPort  Side=Left
  Fd : PMIOPort  Port=2  Side=Right
  wires:
  Wind Speed/1 -> Simulink-PS Converter/1
  connections:
  AirDragForce/RConn1 -- PS Add1/LConn2
  PS Product1/LConn2 -- PS Add1/RConn1
  PS Add2/LConn2 -- Simulink-PS Converter/RConn1
  PS Product/LConn1 -- PS Product/LConn2 -- PS Add2/RConn1
  PS Product1/LConn1 -- Sign/RConn1
  Sign Change/RConn1 -- Fd/RConn1
  AirDragForce/LConn1 -- PS Product/RConn1
  PS Add1/LConn1 -- RollingResistance/RConn1
  Mv*cr1/RConn1 -- RollingResistance/LConn2
  Sign/LConn1 -- Dead Zone/RConn1
  RollingResistance/LConn1 -- Mv*cr2/RConn1
  PS Product1/RConn1 -- Sign Change/LConn1
  Dead Zone/LConn1 -- PS Add2/LConn1 -- v/RConn1 -- Mv*cr2/LConn1

== system IPMSMAxleDriveEV_fihPedals/Vehicle Dynamics/Gravity ==
  Incline : Inport
  GravitationalForce : fl_lib/Physical Signals/Functions/PS Gain  gain=-1 N
  Mv*g : fl_lib/Physical Signals/Functions/PS Gain  gain=Mv*g
  Simulink-PS Converter1 : nesl_utility/Simulink-PS Converter  PhysicalDomain=network_engine_domain  SubClassName=ps_input  LeftPortType=input  RightPortType=output  PseudoPeriodic=off  Frequencies=[]  NoiseDistribution=none  NoiseParameters=[]  Unit=rad  AffineConversion=off  FilteringAndDerivatives=zero  SimscapeFilterOrder=1  InputFilterTimeConstant=0.001  UdotUserProvided=1
  deg->rad : Gain  Gain=pi/180
  sin : fl_lib/Physical Signals/Functions/PS Math Function  fcn_choice=1  v=1
  Fg : PMIOPort  Side=Right
  wires:
  Incline/1 -> deg->rad/1
  deg->rad/1 -> Simulink-PS Converter1/1
  connections:
  Simulink-PS Converter1/RConn1 -- sin/LConn1
  Mv*g/LConn1 -- sin/RConn1
  Mv*g/RConn1 -- GravitationalForce/LConn1
  GravitationalForce/RConn1 -- Fg/RConn1

== system IPMSMAxleDriveEV_fihPedals/Vehicle Dynamics/Sensor Vehicle Speed ==
  MTRef15 : fl_lib/Mechanical/Translational Elements/Mechanical Translational Reference
  PS Terminator : fl_lib/Physical Signals/Sinks/PS Terminator
  Translational Motion Sensor : fl_lib/Mechanical/Mechanical Sensors/Ideal Translational Motion Sensor  reference=foundation.enum.MeasurementReference.difference  acceleration_port=false  velocity_port=true  position_port=true  offset=0 m
  Conn1 : PMIOPort  Side=Left
  Conn2 : PMIOPort  Port=2  Side=Right
  connections:
  Translational Motion Sensor/LConn1 -- Conn1/RConn1
  Translational Motion Sensor/RConn1 -- MTRef15/LConn1
  Translational Motion Sensor/RConn2 -- Conn2/RConn1
  Translational Motion Sensor/RConn3 -- PS Terminator/LConn1

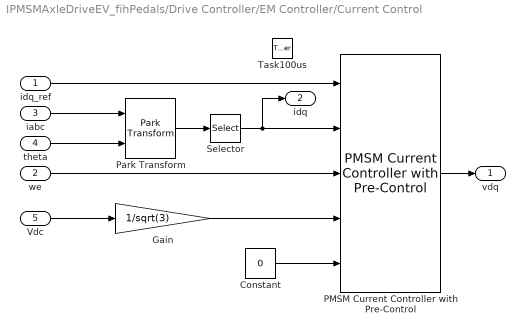
== system IPMSMAxleDriveEV_fihPedals/Drive Controller/EM Controller/Current Control ==
  idq_ref : Inport
  we : Inport  Port=2
  iabc : Inport  Port=3
  theta : Inport  Port=4
  Vdc : Inport  Port=5
  Task100us : TriggerPort  TriggerType=function-call  VariantControl=Variant  PortDimensions=1
  Constant : Constant  Value=0  SampleTime=-1
  Gain : Gain  Gain=1/sqrt(3)
  PMSM Current Controller with Pre-Control : eePmsmCurrentController/PMSM Current Controller with Pre-Control  Kp_id=Kp_id  Ki_id=Ki_id  Kaw_id=1  Kp_iq=Kp_iq  Ki_iq=Ki_iq  Kaw_iq=1  Ts=-1  Tsd=Tsi  AxisPrio=Q-axis  ActZC=on  ActFF=on  idVect=[-200, 0, 200]  iqVect=[-200, 0, 200]  LdMatrix=Ld * ones(3, 3)  LqMatrix=Lq * ones(3, 3)  psimMatrix=psim * ones(3, 3)
  Park Transform : eeTransforms/Park Transform  AxisAlignment=Q-axis  PowerInvariant=off
  Selector : Selector  InputPortWidth=3  IndexOptions=Index vector (dialog)  Indices=[1 2]  OutputSizes=1
  vdq : Outport  VectorParamsAs1DForOutWhenUnconnected=off
  idq : Outport  Port=2  VectorParamsAs1DForOutWhenUnconnected=off
  wires:
  Selector/1 -> idq/1, PMSM Current Controller with Pre-Control/2
  Vdc/1 -> Gain/1
  iabc/1 -> Park Transform/1
  we/1 -> PMSM Current Controller with Pre-Control/3
  Park Transform/1 -> Selector/1
  idq_ref/1 -> PMSM Current Controller with Pre-Control/1
  Constant/1 -> PMSM Current Controller with Pre-Control/5
  theta/1 -> Park Transform/2
  Gain/1 -> PMSM Current Controller with Pre-Control/4
  PMSM Current Controller with Pre-Control/1 -> vdq/1

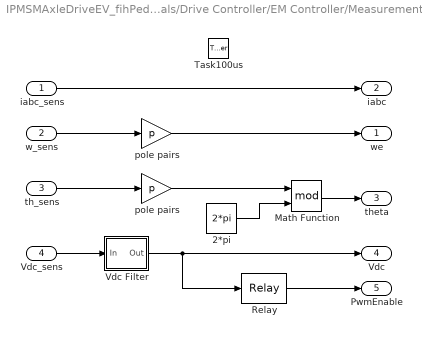
== system IPMSMAxleDriveEV_fihPedals/Drive Controller/EM Controller/Measurements ==
  iabc_sens : Inport
  w_sens : Inport  Port=2
  th_sens : Inport  Port=3
  Vdc_sens : Inport  Port=4
  Task100us : TriggerPort  TriggerType=function-call  VariantControl=Variant  PortDimensions=1
  2*pi : Constant  Value=2*pi  SampleTime=-1
  Math Function : Math  Operator=mod  SignedPower=on
  Relay : Relay  OnSwitchValue=VDC_VECT(1)  OffSwitchValue=0.5*VDC_VECT(1)
  Vdc Filter : Subsystem  mask(Discrete first-order filter (Low-pass)){T=0.01, Ts=1e-4}
      mask prompts: T "Time constant (s):"; Ts "Sample time (s):"
      mask help: This block implements a discrete low-pass filter. To calculate the coefficients, the block discretises a continuous low-pass filter using the Tustin method.
      mask init:
      | num = [ Ts/(2*T + Ts), Ts/(2*T + Ts)];
      | den = [ 1, -(2*T - Ts)/(2*T + Ts)];
  pole pairs : Gain  Gain=p
  "pole pairs " : Gain  Gain=p
  we : Outport  VectorParamsAs1DForOutWhenUnconnected=off
  iabc : Outport  Port=2  VectorParamsAs1DForOutWhenUnconnected=off
  theta : Outport  Port=3  VectorParamsAs1DForOutWhenUnconnected=off
  Vdc : Outport  Port=4  VectorParamsAs1DForOutWhenUnconnected=off
  PwmEnable : Outport  Port=5  VectorParamsAs1DForOutWhenUnconnected=off
  wires:
  pole pairs/1 -> we/1
  th_sens/1 -> "pole pairs "/1
  w_sens/1 -> pole pairs/1
  iabc_sens/1 -> iabc/1
  2*pi/1 -> Math Function/2
  Math Function/1 -> theta/1
  "pole pairs "/1 -> Math Function/1
  Vdc_sens/1 -> Vdc Filter/1(In)
  Relay/1 -> PwmEnable/1
  Vdc Filter/1(Out) -> Relay/1, Vdc/1

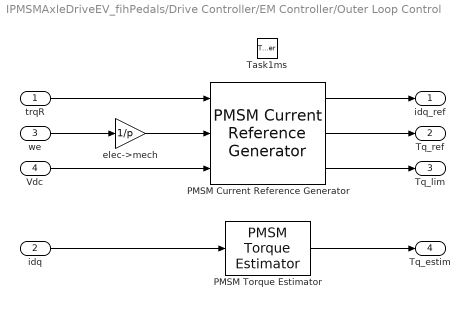
== system IPMSMAxleDriveEV_fihPedals/Drive Controller/EM Controller/Outer Loop Control ==
  trqR : Inport
  idq : Inport  Port=2
  we : Inport  Port=3
  Vdc : Inport  Port=4
  Task1ms : TriggerPort  TriggerType=function-call  VariantControl=Variant  PortDimensions=1
  PMSM Current Reference Generator : eePmsmCurrentReferenceGen/PMSM Current Reference Generator  Vnom=Vnom  Pmax=Pmax  Tmax=Tmax  Ts=-1  RefType=Lookup-table based  rpmVec=RPM_VECT  TqVec=TQ_VECT  VdcVec=VDC_VECT  PWMMode=SVM: space vector modulation  ModFactor=1  idMatrix=ID_MAP  iqMatrix=IQ_MAP  p=8  psim=0.04  Ld=0.00024  Lq=0.00029  Rs=0.01  RefExpEnable=0
  PMSM Torque Estimator : eePmsmTorqueEstimator/PMSM Torque Estimator  ParamType=Constant parameters  p=p  idVect=[-200, 200]  iqVect=[-200, 200]  LdMatrix=0.0002 * ones(2, 2)  LqMatrix=0.0002 * ones(2, 2)  psimMatrix=0.04 * ones(2, 2)  Ld=Ld  Lq=Lq  psim=psim  Ts=-1
  elec->mech : Gain  Gain=1/p
  idq_ref : Outport  VectorParamsAs1DForOutWhenUnconnected=off
  Tq_ref : Outport  Port=2  VectorParamsAs1DForOutWhenUnconnected=off
  Tq_lim : Outport  Port=3  VectorParamsAs1DForOutWhenUnconnected=off
  Tq_estim : Outport  Port=4  VectorParamsAs1DForOutWhenUnconnected=off
  wires:
  idq/1 -> PMSM Torque Estimator/1
  PMSM Current Reference Generator/2 -> Tq_ref/1
  PMSM Current Reference Generator/1 -> idq_ref/1
  Vdc/1 -> PMSM Current Reference Generator/3
  elec->mech/1 -> PMSM Current Reference Generator/2
  trqR/1 -> PMSM Current Reference Generator/1
  PMSM Current Reference Generator/3 -> Tq_lim/1
  we/1 -> elec->mech/1
  PMSM Torque Estimator/1 -> Tq_estim/1

== system IPMSMAxleDriveEV_fihPedals/Drive Controller/EM Controller/Measurements/Vdc Filter ==
  In : Inport
  Discrete Transfer Fcn : DiscreteTransferFcn  Numerator=num  Denominator=den
  Out : Outport  VectorParamsAs1DForOutWhenUnconnected=off
  wires:
  In/1 -> Discrete Transfer Fcn/1
  Discrete Transfer Fcn/1 -> Out/1

== stateflow chart IPMSMAxleDriveEV_fihPedals/Drive Controller/EM Controller/Task Scheduler ==
  (default) -> (junction 23) : CLK_50us
  (junction 23) -> (junction 17)
  (junction 17) -> (junction 22) [order 2]
  (junction 17) -> (junction 22) [order 1] : [cnt%%2==0]{Task_100us_1;}
  (junction 22) -> (junction 18) [order 2]
  (junction 22) -> (junction 18) [order 1] : [cnt%%2==0]{Task_100us_2;}
  (junction 18) -> (junction 37) [order 2]
  (junction 18) -> (junction 37) [order 1] : [cnt%%20==0]{Task_1ms_1;}
  (junction 37) -> (junction 43) [order 2]
  (junction 37) -> (junction 35) [order 1] : [1]{cnt++;}
  data: cnt local int32
  events: Task_100us_1 output FUNCTION_CALL_EVENT; Task_100us_2 output FUNCTION_CALL_EVENT; Task_1ms_1 output FUNCTION_CALL_EVENT; CLK_50us input FUNCTION_CALL_EVENT
